simulink model "s_c_nbe_m32k"  (R2018a)
settings: Solver=VariableStepDiscrete  StartTime=0.0  StopTime=1000  RelTol=1e-3
undefined symbols (not defined in the file): fft_stages, n_taps, output_bits, pfb_coeff_gen_calc, xengbits
libraries: xbsIndex_r4 x23714, casper_library_misc x17, xps_library x4, casper_library_scopes x4, xbsReplacements_r4 x4
(part 4 of 171)

== system s_c_nbe_m32k/DDC ==
  note: DDS 18.17
  note: Mixer
  note: Filter
  sync : Inport
  dvalid : Inport  Port=2
  pol0_data : Inport  Port=3
  osc0 : Inport  Port=4
  pol1_data : Inport  Port=5
  osc1 : Inport  Port=6
  Assert : xbsIndex_r4/Assert  assert_type=on  type_source=Explicitly  gui_display_data_type=Boolean  arith_type=Boolean  n_bits=16  bin_pt=14  preci_type=Single  exp_width=8  frac_width=24  assert_rate=off  rate_source=Explicitly  period=1  output_port=on  block_type=assert
  Concat : xbsIndex_r4/Concat  num_inputs=2  dbl_ovrd=off  block_type=concat
  Concat1 : xbsIndex_r4/Concat  num_inputs=2  dbl_ovrd=off  block_type=concat
  Constant : xbsIndex_r4/Constant  const=0  gui_display_data_type=Fixed-point  arith_type=Unsigned  n_bits=1  bin_pt=0  preci_type=Single  exp_width=8  frac_width=24  explicit_period=on  period=1  equ=P=C  opselect=C  inp2=PCIN>>17  opr=+  inp1=P  carry=CIN  dbl_ovrd=off  block_type=constant
  Counter1 : xbsIndex_r4/Counter  cnt_type=Free Running  cnt_to=Inf  operation=Up  start_count=0  cnt_by_val=1  arith_type=Unsigned  n_bits=8  bin_pt=0  load_pin=off  rst=on  en=on  explicit_period=on  period=1  use_behavioral_HDL=off  implementation=DSP48  dbl_ovrd=off  block_type=counter
      settings: block_version=11.4
  Counter3 : xbsIndex_r4/Counter  cnt_type=Free Running  cnt_to=Inf  operation=Up  start_count=0  cnt_by_val=1  arith_type=Unsigned  n_bits=8  bin_pt=0  load_pin=off  rst=on  en=on  explicit_period=on  period=1  use_behavioral_HDL=off  implementation=DSP48  dbl_ovrd=off  block_type=counter
      settings: block_version=11.4
  Delay1 : xbsIndex_r4/Delay  rst=off  infoeditControl=Selection of Reset will increase slice count due to use of real FFs and instead of SRLs  en=off  latency=12  reg_retiming=off  dbl_ovrd=off  block_type=delay
  Delay2 : xbsIndex_r4/Delay  rst=off  infoeditControl=Selection of Reset will increase slice count due to use of real FFs and instead of SRLs  en=off  latency=12  reg_retiming=off  dbl_ovrd=off  block_type=delay
  Delay3 : xbsIndex_r4/Delay  rst=off  infoeditControl=Selection of Reset will increase slice count due to use of real FFs and instead of SRLs  en=off  latency=1  reg_retiming=off  dbl_ovrd=off  block_type=delay
      settings: infoedit=Hardware notes: A delay line is a chain, each link of which is an SRL16 or SRL32 followed by a flip-flop.
  Delay5 : xbsIndex_r4/Delay  rst=off  infoeditControl=Selection of Reset will increase slice count due to use of real FFs and instead of SRLs  en=off  latency=1  reg_retiming=off  dbl_ovrd=off  block_type=delay
      settings: infoedit=Hardware notes: A delay line is a chain, each link of which is an SRL16 or SRL32 followed by a flip-flop.
  Delay7 : xbsIndex_r4/Delay  rst=off  infoeditControl=Selection of Reset will increase slice count due to use of real FFs and instead of SRLs  en=off  latency=1  reg_retiming=off  dbl_ovrd=off  block_type=delay
      settings: infoedit=Hardware notes: A delay line is a chain, each link of which is an SRL16 or SRL32 followed by a flip-flop.
  Inverter : xbsIndex_r4/Inverter  en=off  latency=0  dbl_ovrd=off  block_type=inv
  Logical : xbsIndex_r4/Logical  Commented=on  logical_function=OR  inputs=2  en=off  latency=0  precision=Full  arith_type=Unsigned  n_bits=16  bin_pt=0  align_bp=on  dbl_ovrd=off  block_type=logical
  Register1 : xbsIndex_r4/Register  init=0  rst=on  en=on  dbl_ovrd=off  block_type=register
  bus_expand : Subsystem  mask(bus_expand){mode=divisions of equal size, outputNum=2, outputWidth=1, outputBinaryPt=0, outputArithmeticType=2, show_format=off, outputToWorkspace=off, variablePrefix=out, outputToModelAsWell=on}
      mask prompts: outputNum "Number of outputs:"; outputWidth "Output width:"; outputBinaryPt "Output binary point position:"; outputArithmeticType "Output arithmetic type (ufix=0, fix=1, bool=2):"; show_format "Print format string?"; outputToWorkspace "Output to workspace?"; variablePrefix "Variable name prefix:"; outputToModelAsWell "Output to model as well?"
      mask help:
      | Expands a 'bus' made using a bus_create or Xilinx
      | concat block.
      | The input will be divided into the specified number
      | of outputs with the specified arithmetic types.
      | Divisions are made from most significant bit.
      mask init: same as s_c_nbe_m32k/bus_expand1
      settings: AttributesFormatString=2 outputs
      mask TypeOptions mode: divisions of equal size | divisions of arbitrary size
      mask Callback mode: bus_expand_callback();
      mask Callback outputWidth: bus_expand_callback();
      mask Callback outputToWorkspace: bus_expand_callback();
  bus_expand10 : Subsystem  mask(bus_expand){mode=divisions of equal size, outputNum=16, outputWidth=18, outputBinaryPt=17, outputArithmeticType=1, show_format=off, outputToWorkspace=off, variablePrefix=Sin, outputToModelAsWell=off}
      mask prompts: outputNum "Number of outputs:"; outputWidth "Output width:"; outputBinaryPt "Output binary point position:"; outputArithmeticType "Output arithmetic type (ufix=0, fix=1, bool=2):"; show_format "Print format string?"; outputToWorkspace "Output to workspace?"; variablePrefix "Variable name prefix:"; outputToModelAsWell "Output to model as well?"
      mask help:
      | Expands a 'bus' made using a bus_create or Xilinx
      | concat block.
      | The input will be divided into the specified number
      | of outputs with the specified arithmetic types.
      | Divisions are made from most significant bit.
      mask init: same as s_c_nbe_m32k/bus_expand1
      settings: AttributesFormatString=16 outputs
      mask TypeOptions mode: divisions of equal size | divisions of arbitrary size
      mask Callback mode: bus_expand_callback();
      mask Callback outputWidth: bus_expand_callback();
      mask Callback outputToWorkspace: bus_expand_callback();
  bus_expand5 : Subsystem  mask(bus_expand){mode=divisions of equal size, outputNum=16, outputWidth=18, outputBinaryPt=17, outputArithmeticType=1, show_format=off, outputToWorkspace=off, variablePrefix=Sin, outputToModelAsWell=off}
      mask prompts: outputNum "Number of outputs:"; outputWidth "Output width:"; outputBinaryPt "Output binary point position:"; outputArithmeticType "Output arithmetic type (ufix=0, fix=1, bool=2):"; show_format "Print format string?"; outputToWorkspace "Output to workspace?"; variablePrefix "Variable name prefix:"; outputToModelAsWell "Output to model as well?"
      mask help:
      | Expands a 'bus' made using a bus_create or Xilinx
      | concat block.
      | The input will be divided into the specified number
      | of outputs with the specified arithmetic types.
      | Divisions are made from most significant bit.
      mask init: same as s_c_nbe_m32k/bus_expand1
      settings: AttributesFormatString=16 outputs
      mask TypeOptions mode: divisions of equal size | divisions of arbitrary size
      mask Callback mode: bus_expand_callback();
      mask Callback outputWidth: bus_expand_callback();
      mask Callback outputToWorkspace: bus_expand_callback();
  bus_expand6 : Subsystem  mask(bus_expand){mode=divisions of equal size, outputNum=16, outputWidth=18, outputBinaryPt=17, outputArithmeticType=1, show_format=off, outputToWorkspace=off, variablePrefix=Sin, outputToModelAsWell=off}
      mask prompts: outputNum "Number of outputs:"; outputWidth "Output width:"; outputBinaryPt "Output binary point position:"; outputArithmeticType "Output arithmetic type (ufix=0, fix=1, bool=2):"; show_format "Print format string?"; outputToWorkspace "Output to workspace?"; variablePrefix "Variable name prefix:"; outputToModelAsWell "Output to model as well?"
      mask help:
      | Expands a 'bus' made using a bus_create or Xilinx
      | concat block.
      | The input will be divided into the specified number
      | of outputs with the specified arithmetic types.
      | Divisions are made from most significant bit.
      mask init: same as s_c_nbe_m32k/bus_expand1
      settings: AttributesFormatString=16 outputs
      mask TypeOptions mode: divisions of equal size | divisions of arbitrary size
      mask Callback mode: bus_expand_callback();
      mask Callback outputWidth: bus_expand_callback();
      mask Callback outputToWorkspace: bus_expand_callback();
  bus_expand9 : Subsystem  mask(bus_expand){mode=divisions of equal size, outputNum=16, outputWidth=18, outputBinaryPt=17, outputArithmeticType=1, show_format=off, outputToWorkspace=off, variablePrefix=Sin, outputToModelAsWell=off}
      mask prompts: outputNum "Number of outputs:"; outputWidth "Output width:"; outputBinaryPt "Output binary point position:"; outputArithmeticType "Output arithmetic type (ufix=0, fix=1, bool=2):"; show_format "Print format string?"; outputToWorkspace "Output to workspace?"; variablePrefix "Variable name prefix:"; outputToModelAsWell "Output to model as well?"
      mask help:
      | Expands a 'bus' made using a bus_create or Xilinx
      | concat block.
      | The input will be divided into the specified number
      | of outputs with the specified arithmetic types.
      | Divisions are made from most significant bit.
      mask init: same as s_c_nbe_m32k/bus_expand1
      settings: AttributesFormatString=16 outputs
      mask TypeOptions mode: divisions of equal size | divisions of arbitrary size
      mask Callback mode: bus_expand_callback();
      mask Callback outputWidth: bus_expand_callback();
      mask Callback outputToWorkspace: bus_expand_callback();
  bus_mult : Subsystem  mask(bus_mult){n_bits_a=[10,10,10,10,10,10,10,10], bin_pt_a=9, type_a=1, cmplx_a=on, n_bits_b=[18,18,18,18,18,18,18,18], bin_pt_b=17, type_b=1, cmplx_b=on, misc=on, floating_point=off, float_type=single, input_vec_a=1, input_vec_b=1, frac_width=19, exp_width=6, n_bits_out=18, bin_pt_out=17, type_out=1, quantization=1, overflow=0, mult_latency=7, add_latency=7, conv_latency=7, max_fanout=1, fan_latency=3, multiplier_implementation=embedded multiplier core, pipeline_cmult_en=off, pipeline_latency=0}
      mask prompts: n_bits_a "a input bit widths"; bin_pt_a "a input binary points"; type_a "a input type (Unsigned=0, Signed=1)"; cmplx_a "a input complex"; n_bits_b "b input bit widths"; bin_pt_b "b input binary points"; type_b "b input type (Unsigned=0, Signed=1)"; cmplx_b "b input complex"; misc "misc support"; floating_point "floating point"; float_type "float type"; input_vec_a "a input vector in bus"; input_vec_b "b input vector in bus"; frac_width "fraction width"; exp_width "exponent width"; n_bits_out "output bit widths"; bin_pt_out "output binary points"; type_out "output type (Unsigned=0, Signed=1)"; quantization "quantization strategy (Truncate=0, Round  (unbiased: +/- Inf)=1)"; overflow "overflow strategy (Wrap=0, Saturate=1, Flag as error=2)"; mult_latency "multiplier latency"; add_latency "adder latency"; conv_latency "convert latency"; max_fanout "limit fanout to ?"; fan_latency "fanout register latency"; multiplier_implementation "multiplier implementation"; pipeline_cmult_en "pipeline complex mult"; pipeline_latency "pipeline latency"
      mask help: Multiply components of two busses
      mask init:
      | bus_mult_init(gcb, ...
      |     'n_bits_a', n_bits_a, ...
      |     'bin_pt_a', bin_pt_a, ...
      |     'type_a', type_a, ...
      |     'cmplx_a', cmplx_a, ...
      |     'n_bits_b', n_bits_b, ...
      |     'bin_pt_b', bin_pt_b, ...
      |     'type_b', type_b, ...
      |     'cmplx_b', cmplx_b, ...
      |     'n_bits_out', n_bits_out, ...
      |     'bin_pt_out', bin_pt_out, ...
      |     'type_out', type_out, ...
      |     'floating_point', floating_point, ...
      |     'float_type', float_type, ...
      |     'exp_width', exp_width, ...
      |     'input_vec_a', input_vec_a, ...
      |     'input_vec_b', input_vec_b, ...
      |     'frac_width', frac_width, ...         
      |     'quantization', quantization, ...
      |     'overflow', overflow, ...
      |     'mult_latency', mult_latency, ...
      |     'add_latency', add_latency, ...
      |     'conv_latency', conv_latency, ...
      |     'max_fanout', max_fanout, ...
      |     'pipeline_cmult_en', pipeline_cmult_en, ...
      |     'pipeline_latency', pipeline_latency, ...
      |     'fan_latency', fan_latency, ...
      |     'multiplier_implementation', multiplier_implementation, ...
      |     'misc', misc);
      mask Callback floating_point:
      | onoff = get_param(gcb, 'floating_point');
      | if strcmp(onoff,'on')
      |     enable_fixpt = 'off'
      |     set_param_state(gcb, 'float_type', 'on')
      | 
      |     set_param_state(gcb, 'input_vec_a', 'on')
      |     set_param_state(gcb, 'input_vec_b', 'on')
      | 
      |     f_type = get_param(gcb, 'float_type')
      |     if strcmp(f_type,'custom')
      |         set_param_state(gcb, 'exp_width', 'on')
      |         set_param_state(gcb, 'frac_width', 'on')
      |     else
      |         set_param_state(gcb, 'exp_width', 'off')
      |         set_param_state(gcb, 'frac_width', 'off')
      |     end
      | 
      | else
      |     enable_fixpt = 'on'
      |     set_param_state(gcb, 'float_type', 'off')
      |     set_param_state(gcb, 'exp_width', 'off')
      |     set_param_state(gcb, 'frac_width', 'off')
      |     set_param_state(gcb, 'input_vec_a', 'off')
      |     set_param_state(gcb, 'input_vec_b', 'off')
      | end
      | 
      | set_param_state(gcb, 'n_bits_a', enable_fixpt)
      | set_param_state(gcb, 'bin_pt_a', enable_fixpt)
      | set_param_state(gcb, 'type_a', enable_fixpt)
      | set_param_state(gcb, 'n_bits_b', enable_fixpt)
      | set_param_state(gcb, 'bin_pt_b', enable_fixpt)
      | set_param_state(gcb, 'type_b', enable_fixpt)
      | 
      | set_param_state(gcb, 'n_bits_out', enable_fixpt)
      | set_param_state(gcb, 'bin_pt_out', enable_fixpt)
      | set_param_state(gcb, 'type_out', enable_fixpt)
      | set_param_state(gcb, 'quantization', enable_fixpt)
      | set_param_state(gcb, 'overflow', enable_fixpt)
      mask TypeOptions float_type: single | custom
      mask Callback float_type:
      | f_type = get_param(gcb, 'float_type')
      | if strcmp(f_type,'custom')
      |     set_param_state(gcb, 'exp_width', 'on')
      |     set_param_state(gcb, 'frac_width', 'on')
      | else
      |     set_param_state(gcb, 'exp_width', 'off')
      |     set_param_state(gcb, 'frac_width', 'off')
      | end
      mask TypeOptions multiplier_implementation: behavioral HDL | standard core | embedded multiplier core
      mask Callback pipeline_cmult_en:
      | pipeline_en = get_param(gcb, 'pipeline_cmult_en');
      | if strcmp(pipeline_en,'on')
      | 
      |     set_param_state(gcb, 'pipeline_latency', 'on')
      | else
      |     set_param_state(gcb, 'pipeline_latency', 'off')
      | end
  bus_mult1 : Subsystem  mask(bus_mult){n_bits_a=[10,10,10,10,10,10,10,10], bin_pt_a=9, type_a=1, cmplx_a=on, n_bits_b=[18,18,18,18,18,18,18,18], bin_pt_b=17, type_b=1, cmplx_b=on, misc=off, floating_point=off, float_type=single, input_vec_a=1, input_vec_b=1, frac_width=19, exp_width=6, n_bits_out=18, bin_pt_out=17, type_out=1, quantization=1, overflow=0, mult_latency=7, add_latency=7, conv_latency=7, max_fanout=1, fan_latency=3, multiplier_implementation=embedded multiplier core, pipeline_cmult_en=off, pipeline_latency=0}
      mask prompts: n_bits_a "a input bit widths"; bin_pt_a "a input binary points"; type_a "a input type (Unsigned=0, Signed=1)"; cmplx_a "a input complex"; n_bits_b "b input bit widths"; bin_pt_b "b input binary points"; type_b "b input type (Unsigned=0, Signed=1)"; cmplx_b "b input complex"; misc "misc support"; floating_point "floating point"; float_type "float type"; input_vec_a "a input vector in bus"; input_vec_b "b input vector in bus"; frac_width "fraction width"; exp_width "exponent width"; n_bits_out "output bit widths"; bin_pt_out "output binary points"; type_out "output type (Unsigned=0, Signed=1)"; quantization "quantization strategy (Truncate=0, Round  (unbiased: +/- Inf)=1)"; overflow "overflow strategy (Wrap=0, Saturate=1, Flag as error=2)"; mult_latency "multiplier latency"; add_latency "adder latency"; conv_latency "convert latency"; max_fanout "limit fanout to ?"; fan_latency "fanout register latency"; multiplier_implementation "multiplier implementation"; pipeline_cmult_en "pipeline complex mult"; pipeline_latency "pipeline latency"
      mask help: Multiply components of two busses
      mask init: same as s_c_nbe_m32k/DDC/bus_mult
      mask Callback floating_point:
      | onoff = get_param(gcb, 'floating_point');
      | if strcmp(onoff,'on')
      |     enable_fixpt = 'off'
      |     set_param_state(gcb, 'float_type', 'on')
      | 
      |     set_param_state(gcb, 'input_vec_a', 'on')
      |     set_param_state(gcb, 'input_vec_b', 'on')
      | 
      |     f_type = get_param(gcb, 'float_type')
      |     if strcmp(f_type,'custom')
      |         set_param_state(gcb, 'exp_width', 'on')
      |         set_param_state(gcb, 'frac_width', 'on')
      |     else
      |         set_param_state(gcb, 'exp_width', 'off')
      |         set_param_state(gcb, 'frac_width', 'off')
      |     end
      | 
      | else
      |     enable_fixpt = 'on'
      |     set_param_state(gcb, 'float_type', 'off')
      |     set_param_state(gcb, 'exp_width', 'off')
      |     set_param_state(gcb, 'frac_width', 'off')
      |     set_param_state(gcb, 'input_vec_a', 'off')
      |     set_param_state(gcb, 'input_vec_b', 'off')
      | end
      | 
      | set_param_state(gcb, 'n_bits_a', enable_fixpt)
      | set_param_state(gcb, 'bin_pt_a', enable_fixpt)
      | set_param_state(gcb, 'type_a', enable_fixpt)
      | set_param_state(gcb, 'n_bits_b', enable_fixpt)
      | set_param_state(gcb, 'bin_pt_b', enable_fixpt)
      | set_param_state(gcb, 'type_b', enable_fixpt)
      | 
      | set_param_state(gcb, 'n_bits_out', enable_fixpt)
      | set_param_state(gcb, 'bin_pt_out', enable_fixpt)
      | set_param_state(gcb, 'type_out', enable_fixpt)
      | set_param_state(gcb, 'quantization', enable_fixpt)
      | set_param_state(gcb, 'overflow', enable_fixpt)
      mask TypeOptions float_type: single | custom
      mask Callback float_type:
      | f_type = get_param(gcb, 'float_type')
      | if strcmp(f_type,'custom')
      |     set_param_state(gcb, 'exp_width', 'on')
      |     set_param_state(gcb, 'frac_width', 'on')
      | else
      |     set_param_state(gcb, 'exp_width', 'off')
      |     set_param_state(gcb, 'frac_width', 'off')
      | end
      mask TypeOptions multiplier_implementation: behavioral HDL | standard core | embedded multiplier core
      mask Callback pipeline_cmult_en:
      | pipeline_en = get_param(gcb, 'pipeline_cmult_en');
      | if strcmp(pipeline_en,'on')
      | 
      |     set_param_state(gcb, 'pipeline_latency', 'on')
      | else
      |     set_param_state(gcb, 'pipeline_latency', 'off')
      | end
  convert_of : Subsystem  Commented=on  AncestorBlock=casper_library_misc/convert_of  mask(convert_of){bit_width_i=44, binary_point_i=34, bit_width_o=18, binary_point_o=17, latency=2, overflow=Saturate, quantization=Round  (unbiased: +/- Inf)}
      mask prompts: bit_width_i "Bit Width In"; binary_point_i "Binary Point In"; bit_width_o "Bit Width Out"; binary_point_o "Binary Point Out"; overflow "Overflow Behaviour"; quantization "Quantization Behaviour"
      mask help:
      | Converts from one 2's complement bit-width
      | and/or binary point position to another.
      | Includes underflow/overflow indicator.
      mask init:
      | convert_of_init(gcb, ...
      |     'bit_width_i', bit_width_i, ...
      |     'binary_point_i', binary_point_i, ...
      |     'bit_width_o', bit_width_o, ...
      |     'binary_point_o', binary_point_o, ...
      |     'latency', latency, ...
      |     'overflow', overflow, ...
      |     'quantization', quantization);
      settings: AttributesFormatString=[44,34]->[18,17]
      mask TypeOptions overflow: Wrap | Saturate | Error
      mask TypeOptions quantization: Truncate | Round  (unbiased: +/- Inf) | Round  (unbiased: even values)
  convert_of1 : Subsystem  Commented=on  AncestorBlock=casper_library_misc/convert_of  mask(convert_of){bit_width_i=44, binary_point_i=34, bit_width_o=18, binary_point_o=17, latency=2, overflow=Saturate, quantization=Round  (unbiased: +/- Inf)}
      mask prompts: bit_width_i "Bit Width In"; binary_point_i "Binary Point In"; bit_width_o "Bit Width Out"; binary_point_o "Binary Point Out"; overflow "Overflow Behaviour"; quantization "Quantization Behaviour"
      mask help:
      | Converts from one 2's complement bit-width
      | and/or binary point position to another.
      | Includes underflow/overflow indicator.
      mask init: same as s_c_nbe_m32k/DDC/convert_of
      settings: AttributesFormatString=[44,34]->[18,17]
      mask TypeOptions overflow: Wrap | Saturate | Error
      mask TypeOptions quantization: Truncate | Round  (unbiased: +/- Inf) | Round  (unbiased: even values)
  ddc_in_sync_cnt : Subsystem  Tag=xps:sw_reg  AncestorBlock=xps_library/Memory/software_register  mask(swreg){io_dir=To Processor, io_delay=0, init_val=0, sample_period=1, names=reg, bitwidths=8, bin_pts=0, arith_types=0, sim_port=off, show_format=on}
      mask prompts: io_dir "I/O direction"; io_delay "I/O delay"; init_val "Initial Value"; sample_period "Sample period"; names "Bitfield names [msb...lsb]"; bitwidths "Bitfield widths"; bin_pts "Bitfield binary pts"; arith_types "Bitfield types, ufix=0, fix=1, bool=2"; sim_port "Provide sim input/output?"; show_format "Print format string?"
      mask help: A 32-bit software-accessible register. Can be divided into bitfields of varying widths and types using the fields in the block mask.
      mask init:
      | swreg_init(gcb)
      settings: AttributesFormatString=1output:uf8.0 = 8 bits
      mask TypeOptions io_dir: To Processor | From Processor
      mask Callback io_dir:
      | mask_enables = get_param(gcb, 'MaskEnables');
      | mask_names = get_param(gcb, 'MaskNames');
      | if strcmp(get_param(gcb, 'io_dir'), 'To Processor'),
      |     mask_enables{ismember(mask_names, 'sample_period')} = 'off';
      | else
      |     mask_enables{ismember(mask_names, 'sample_period')} = 'on';
      | end
      | set_param(gcb, 'MaskEnables', mask_enables);
      mask DialogControl ParameterTabVar0 Prompt: Setup
  ddc_out_sync_cnt : Subsystem  Tag=xps:sw_reg  AncestorBlock=xps_library/Memory/software_register  mask(swreg){io_dir=To Processor, io_delay=0, init_val=0, sample_period=1, names=reg, bitwidths=8, bin_pts=0, arith_types=0, sim_port=off, show_format=on}
      mask prompts: io_dir "I/O direction"; io_delay "I/O delay"; init_val "Initial Value"; sample_period "Sample period"; names "Bitfield names [msb...lsb]"; bitwidths "Bitfield widths"; bin_pts "Bitfield binary pts"; arith_types "Bitfield types, ufix=0, fix=1, bool=2"; sim_port "Provide sim input/output?"; show_format "Print format string?"
      mask help: A 32-bit software-accessible register. Can be divided into bitfields of varying widths and types using the fields in the block mask.
      mask init:
      | swreg_init(gcb)
      settings: AttributesFormatString=1output:uf8.0 = 8 bits
      mask TypeOptions io_dir: To Processor | From Processor
      mask Callback io_dir:
      | mask_enables = get_param(gcb, 'MaskEnables');
      | mask_names = get_param(gcb, 'MaskNames');
      | if strcmp(get_param(gcb, 'io_dir'), 'To Processor'),
      |     mask_enables{ismember(mask_names, 'sample_period')} = 'off';
      | else
      |     mask_enables{ismember(mask_names, 'sample_period')} = 'on';
      | end
      | set_param(gcb, 'MaskEnables', mask_enables);
      mask DialogControl ParameterTabVar0 Prompt: Setup
  dec_fir_async1 : Subsystem  Tag=casper:dec_fir_async  AncestorBlock=casper_library_downconverter/dec_fir_async  mask(dec_fir_async){n_inputs=16, coeff=[-0.000309,-0.000234,-0.000315,-0.000409,-0.000513,-0.000626,-0.000747,-0.000870,-0.000994,-0.001113,-0.001222,-0.001316,-0.001388,-0.001433,-0.001444,-0.001415,-0.001343,-0.001221,-0.001046,-0.000817,-0.000533,-0.000195,0.000193,0.000628,0.001100,0.001602,0.002121,0.002645,0.003159,0.003646,0.004091,0.004475,0.004781,0.004993,0.005095,0.005074,0.004920,0.004623,0.004179,0.003589,0.002855,0.001988,0.001000,-0.000089,-0.001258,-0.002478,-0.003716,-0.004939,-0.006108,-0.007182,-0.008120,-0.008882,-0.009426,-0.009715,-0.009715,-0.009394,-0.008727,-0.007696,-0.006289,-0.004503,-0.002341,0.000182,0.003046,0.006221,0.009667,0.013340,0.017186,0.021147,0.025161,0.029161,0.033078,0.036845,0.040394,0.043661,0.046586,0.049113,0.051195,0.052792,0.053875,0.054421,0.054421,0.053875,0.052792,0.051195,0.049113,0.046586,0.043661,0.040394,0.036845,0.033078,0.029161,0.025161,0.021147,0.017186,0.013340,0.009667,0.006221,0.003046,0.000182,-0.002341,-0.004503,-0.006289,-0.007696,-0.008727,-0.009394,-0.009715,-0.009715,-0.009426,-0.008882,-0.008120,-0.007182,-0.006108,-0.004939,-0.003716,-0.002478,-0.001258,-0.000089,0.001000,0.001988,0.002855,0.003589,0.004179,0.004623,0.004920,0.005074,0.005095,0.004993,0.004781,0.004475,0.004091,0.003646,0.003159,0.002645,0.002121,0.001602,0.001100,0.000628,0.000193,-0.000195,-0.000533,-0.000817,-0.001046,-0.001221,-0.001343,-0.001415,-0.001444,-0.001433,-0.001388,-0.001316,-0.001222,-0.001113,-0.000994,-0.000870,-0.000747,-0.000626,-0.000513,-0.000409,-0.000315,-0.000234,-0.000309], output_width=18, output_bp=17, quantization=Round  (unbiased: +/- Inf), add_latency=7, mult_latency=7, conv_latency=7, coeff_bit_width=18, coeff_bin_pt=17, lshift=1, absorb_adders=on, adder_imp=DSP48, async=on, bus_input=off, input_width=0, input_bp=0, input_type=Signed}
      mask prompts: n_inputs "Number of Parallel Streams"; coeff "Coefficients"; output_width "Output bitwidth"; output_bp "Output binary point"; quantization "Quantization Behavior"; add_latency "Add Latency"; mult_latency "Mult Latency"; conv_latency "Convert latency"; coeff_bit_width "Coefficient bitwidth"; coeff_bin_pt "Coefficient binary point"; lshift "Post adder-tree shift"; absorb_adders "Absorb adders into DSP slices"; adder_imp "Adder implementation"; async "Asynchronous ops"; bus_input "Bus input"; input_width "Input bitwidth"; input_bp "Input binary point"; input_type "Input datatype"
      mask help: FIR filter which can handle multiple time samples in parallel and decimates down to 1 time sample. If coefficients are symmetric, will automatically fold before multiplying.
      mask init:
      | dec_fir_async_init(gcb);
      settings: AttributesFormatString=|
      | 160 taps
      | 18_17 r/i
      mask TypeOptions quantization: Truncate | Round  (unbiased: +/- Inf) | Round  (unbiased: Even Values)
      mask TypeOptions adder_imp: Behavioral | Fabric | DSP48
      mask Callback bus_input:
      | onoff = get_param(gcb, 'bus_input');
      | set_param_state(gcb, 'input_width', onoff)
      | set_param_state(gcb, 'input_bp', onoff)
      | set_param_state(gcb, 'input_type', onoff)
      mask TypeOptions input_type: Signed | Unsigned
  dec_fir_async3 : Subsystem  Tag=casper:dec_fir_async  AncestorBlock=casper_library_downconverter/dec_fir_async  mask(dec_fir_async){n_inputs=16, coeff=[-0.000309,-0.000234,-0.000315,-0.000409,-0.000513,-0.000626,-0.000747,-0.000870,-0.000994,-0.001113,-0.001222,-0.001316,-0.001388,-0.001433,-0.001444,-0.001415,-0.001343,-0.001221,-0.001046,-0.000817,-0.000533,-0.000195,0.000193,0.000628,0.001100,0.001602,0.002121,0.002645,0.003159,0.003646,0.004091,0.004475,0.004781,0.004993,0.005095,0.005074,0.004920,0.004623,0.004179,0.003589,0.002855,0.001988,0.001000,-0.000089,-0.001258,-0.002478,-0.003716,-0.004939,-0.006108,-0.007182,-0.008120,-0.008882,-0.009426,-0.009715,-0.009715,-0.009394,-0.008727,-0.007696,-0.006289,-0.004503,-0.002341,0.000182,0.003046,0.006221,0.009667,0.013340,0.017186,0.021147,0.025161,0.029161,0.033078,0.036845,0.040394,0.043661,0.046586,0.049113,0.051195,0.052792,0.053875,0.054421,0.054421,0.053875,0.052792,0.051195,0.049113,0.046586,0.043661,0.040394,0.036845,0.033078,0.029161,0.025161,0.021147,0.017186,0.013340,0.009667,0.006221,0.003046,0.000182,-0.002341,-0.004503,-0.006289,-0.007696,-0.008727,-0.009394,-0.009715,-0.009715,-0.009426,-0.008882,-0.008120,-0.007182,-0.006108,-0.004939,-0.003716,-0.002478,-0.001258,-0.000089,0.001000,0.001988,0.002855,0.003589,0.004179,0.004623,0.004920,0.005074,0.005095,0.004993,0.004781,0.004475,0.004091,0.003646,0.003159,0.002645,0.002121,0.001602,0.001100,0.000628,0.000193,-0.000195,-0.000533,-0.000817,-0.001046,-0.001221,-0.001343,-0.001415,-0.001444,-0.001433,-0.001388,-0.001316,-0.001222,-0.001113,-0.000994,-0.000870,-0.000747,-0.000626,-0.000513,-0.000409,-0.000315,-0.000234,-0.000309], output_width=18, output_bp=17, quantization=Round  (unbiased: +/- Inf), add_latency=7, mult_latency=7, conv_latency=7, coeff_bit_width=18, coeff_bin_pt=17, lshift=1, absorb_adders=on, adder_imp=DSP48, async=on, bus_input=off, input_width=0, input_bp=0, input_type=Signed}
      mask prompts: n_inputs "Number of Parallel Streams"; coeff "Coefficients"; output_width "Output bitwidth"; output_bp "Output binary point"; quantization "Quantization Behavior"; add_latency "Add Latency"; mult_latency "Mult Latency"; conv_latency "Convert latency"; coeff_bit_width "Coefficient bitwidth"; coeff_bin_pt "Coefficient binary point"; lshift "Post adder-tree shift"; absorb_adders "Absorb adders into DSP slices"; adder_imp "Adder implementation"; async "Asynchronous ops"; bus_input "Bus input"; input_width "Input bitwidth"; input_bp "Input binary point"; input_type "Input datatype"
      mask help: FIR filter which can handle multiple time samples in parallel and decimates down to 1 time sample. If coefficients are symmetric, will automatically fold before multiplying.
      mask init:
      | dec_fir_async_init(gcb);
      settings: AttributesFormatString=|
      | 160 taps
      | 18_17 r/i
      mask TypeOptions quantization: Truncate | Round  (unbiased: +/- Inf) | Round  (unbiased: Even Values)
      mask TypeOptions adder_imp: Behavioral | Fabric | DSP48
      mask Callback bus_input:
      | onoff = get_param(gcb, 'bus_input');
      | set_param_state(gcb, 'input_width', onoff)
      | set_param_state(gcb, 'input_bp', onoff)
      | set_param_state(gcb, 'input_type', onoff)
      mask TypeOptions input_type: Signed | Unsigned
  edge_detect2 : Subsystem  mask(edge_detect){edge=Rising, polarity=Active High, x_in=[0 0.08 0.08 0.16 0.16 0.24 0.24 0.32 0.32 0.4], y_in=[-1 -1  1  1  1  1  1  1  1  1], x_out=[0.6 0.68 0.68 0.76 0.76 0.84 0.84 0.92 0.92 1], y_out=[-1 -1  1  1 -1 -1 -1 -1 -1 -1]}
      mask prompts: edge "Edge Type"; polarity "Output Polarity"; x_in "Input X Positions"; y_in "Input Y Positions"; x_out "Output X Positions"; y_out "Output Y Positions"
      mask help: Output is active for one-cycle after each edge of the specified type (i.e. rising, falling or both).
      mask init: same as s_c_nbe_m32k/edge_detect1
      settings: AttributesFormatString=|
      | rising edges
      | active high
      mask Help: Output is active for one-cycle after each edge of the specified type (i.e. rising, falling, or both).  Latency is zero.
      mask TypeOptions edge: Rising | Falling | Both
      mask TypeOptions polarity: Active High | Active Low
      mask Display:
      | plot(x_in_num,0.5+y_in_num*0.2);
      | plot(x_out_num,0.5+y_out_num*0.2);
  edge_detect3 : Subsystem  mask(edge_detect){edge=Rising, polarity=Active High, x_in=[0 0.08 0.08 0.16 0.16 0.24 0.24 0.32 0.32 0.4], y_in=[-1 -1  1  1  1  1  1  1  1  1], x_out=[0.6 0.68 0.68 0.76 0.76 0.84 0.84 0.92 0.92 1], y_out=[-1 -1  1  1 -1 -1 -1 -1 -1 -1]}
      mask prompts: edge "Edge Type"; polarity "Output Polarity"; x_in "Input X Positions"; y_in "Input Y Positions"; x_out "Output X Positions"; y_out "Output Y Positions"
      mask help: Output is active for one-cycle after each edge of the specified type (i.e. rising, falling or both).
      mask init: same as s_c_nbe_m32k/edge_detect1
      settings: AttributesFormatString=|
      | rising edges
      | active high
      mask Help: Output is active for one-cycle after each edge of the specified type (i.e. rising, falling, or both).  Latency is zero.
      mask TypeOptions edge: Rising | Falling | Both
      mask TypeOptions polarity: Active High | Active Low
      mask Display:
      | plot(x_in_num,0.5+y_in_num*0.2);
      | plot(x_out_num,0.5+y_out_num*0.2);
  pipeline21 : Subsystem  Tag=cmac_delinked  mask(pipeline){csp_latency=2}
      mask prompts: csp_latency "Latency"
      mask help:
      | An explicitly laid-out delay line to avoid mapping to SRL16s
      | for use in pipelining to help achieve timing closure.
      mask init:
      | pipeline_init(gcb,'latency',csp_latency);
      settings: AttributesFormatString=Latency = %<latency>
      mask Display:
      | port_label('input', 1, 'd');
      | port_label('output', 1, 'q');
      | disp(['Z^-', num2str(csp_latency)]);
  pipeline22 : Subsystem  Tag=cmac_delinked  mask(pipeline){csp_latency=2}
      mask prompts: csp_latency "Latency"
      mask help:
      | An explicitly laid-out delay line to avoid mapping to SRL16s
      | for use in pipelining to help achieve timing closure.
      mask init:
      | pipeline_init(gcb,'latency',csp_latency);
      settings: AttributesFormatString=Latency = %<latency>
      mask Display:
      | port_label('input', 1, 'd');
      | port_label('output', 1, 'q');
      | disp(['Z^-', num2str(csp_latency)]);
  pipeline39 : Subsystem  Tag=cmac_delinked  mask(pipeline){csp_latency=2}
      mask prompts: csp_latency "Latency"
      mask help:
      | An explicitly laid-out delay line to avoid mapping to SRL16s
      | for use in pipelining to help achieve timing closure.
      mask init:
      | pipeline_init(gcb,'latency',csp_latency);
      settings: AttributesFormatString=Latency = %<latency>
      mask Display:
      | port_label('input', 1, 'd');
      | port_label('output', 1, 'q');
      | disp(['Z^-', num2str(csp_latency)]);
  pipeline40 : Subsystem  Tag=cmac_delinked  mask(pipeline){csp_latency=2}
      mask prompts: csp_latency "Latency"
      mask help:
      | An explicitly laid-out delay line to avoid mapping to SRL16s
      | for use in pipelining to help achieve timing closure.
      mask init:
      | pipeline_init(gcb,'latency',csp_latency);
      settings: AttributesFormatString=Latency = %<latency>
      mask Display:
      | port_label('input', 1, 'd');
      | port_label('output', 1, 'q');
      | disp(['Z^-', num2str(csp_latency)]);
  ri_to_c1 : casper_library_misc/ri_to_c  Commented=on
      settings: SourceProductName=CASPER DSP Blockset
  ddc_sync : Outport
  ddc_pol0 : Outport  Port=2
  ddc_pol1 : Outport  Port=3
  ddc_dv : Outport  Port=4
  ddc_of : Outport  Port=5
  tag scope: dec_dv=global, dec_sync=global, mix_80_0=global, mix_dvalid=global, mix_sync=global
  wires:
  bus_expand/1(msb_out2) -> [mix_sync]
  bus_expand/2(lsb_out1) -> [mix_dvalid]
  Concat/1 -> bus_mult/3(misci)
  bus_mult/2(misco) -> bus_expand/1(bus_in)
  [ddc_sync] -> ddc_sync/1
  [ddc_pol0] -> ddc_pol0/1
  [ddc_pol1] -> ddc_pol1/1
  pol0_data/1 -> bus_mult/1(a)
  osc0/1 -> bus_mult/2(b)
  pol1_data/1 -> bus_mult1/1(a)
  osc1/1 -> bus_mult1/2(b)
  bus_mult/1(a*b) -> [mix_80_0]
  bus_mult1/1(a*b) -> [mix_80_1]
  dvalid/1 -> Concat/2
  sync/1 -> Concat/1
  [cnt_rst] -> pipeline22/1(d)
  Counter1/1 -> ddc_out_sync_cnt/1(out_reg)
  pipeline21/1(q) -> Counter1/2
  pipeline22/1(q) -> Counter1/1
  [ddc_sync] -> pipeline21/1(d)
  [ddc_dvalid] -> ddc_dv/1
  Delay3/1 -> bus_expand5/1(bus_in)
  Delay5/1 -> bus_expand9/1(bus_in)
  bus_expand9/1(msb_out16) -> dec_fir_async1/3(real1)
  bus_expand9/2(out15) -> dec_fir_async1/4(imag1)
  bus_expand9/3(out14) -> dec_fir_async1/5(real2)
  bus_expand9/4(out13) -> dec_fir_async1/6(imag2)
  bus_expand9/5(out12) -> dec_fir_async1/7(real3)
  bus_expand9/6(out11) -> dec_fir_async1/8(imag3)
  bus_expand9/7(out10) -> dec_fir_async1/9(real4)
  bus_expand9/8(out9) -> dec_fir_async1/10(imag4)
  bus_expand9/9(out8) -> dec_fir_async1/11(real5)
  bus_expand9/10(out7) -> dec_fir_async1/12(imag5)
  bus_expand9/11(out6) -> dec_fir_async1/13(real6)
  bus_expand9/12(out5) -> dec_fir_async1/14(imag6)
  bus_expand9/13(out4) -> dec_fir_async1/15(real7)
  bus_expand9/14(out3) -> dec_fir_async1/16(imag7)
  bus_expand9/15(out2) -> dec_fir_async1/17(real8)
  bus_expand9/16(lsb_out1) -> dec_fir_async1/18(imag8)
  bus_expand10/1(msb_out16) -> dec_fir_async1/19(real9)
  bus_expand10/3(out14) -> dec_fir_async1/21(real10)
  bus_expand10/2(out15) -> dec_fir_async1/20(imag9)
  bus_expand10/4(out13) -> dec_fir_async1/22(imag10)
  bus_expand10/5(out12) -> dec_fir_async1/23(real11)
  bus_expand10/7(out10) -> dec_fir_async1/25(real12)
  bus_expand10/6(out11) -> dec_fir_async1/24(imag11)
  bus_expand10/8(out9) -> dec_fir_async1/26(imag12)
  bus_expand10/9(out8) -> dec_fir_async1/27(real13)
  bus_expand10/10(out7) -> dec_fir_async1/28(imag13)
  bus_expand10/11(out6) -> dec_fir_async1/29(real14)
  bus_expand10/12(out5) -> dec_fir_async1/30(imag14)
  bus_expand10/14(out3) -> dec_fir_async1/32(imag15)
  bus_expand10/13(out4) -> dec_fir_async1/31(real15)
  bus_expand10/15(out2) -> dec_fir_async1/33(real16)
  bus_expand10/16(lsb_out1) -> dec_fir_async1/34(imag16)
  dec_fir_async1/2(dout) -> Delay2/1
  [cnt_rst] -> pipeline40/1(d)
  Counter3/1 -> ddc_in_sync_cnt/1(out_reg)
  pipeline39/1(q) -> Counter3/2
  pipeline40/1(q) -> Counter3/1
  [dec_sync] -> pipeline39/1(d)
  [mix_dvalid] -> Register1/3
  Register1/1 -> edge_detect3/1(in), Inverter/1
  edge_detect3/1(out) -> [dec_dv]
  [dec_sync] -> dec_fir_async3/1(sync_in)
  [dec_dv] -> dec_fir_async1/2(dv_in)
  [dec_sync] -> dec_fir_async1/1(sync_in)
  [mix_80_1] -> Delay5/1, bus_expand10/1(bus_in)
  [mix_80_0] -> bus_expand6/1(bus_in), Delay3/1
  edge_detect2/1(out) -> [dec_sync]
  Inverter/1 -> Assert/1
  Assert/1 -> Register1/1
  [mix_sync] -> Delay7/1, Register1/2
  Delay7/1 -> edge_detect2/1(in)
  [ddc_of_pol0] -> Concat1/1
  [ddc_of_pol1] -> Concat1/2
  Concat1/1 -> ddc_of/1
  dec_fir_async3/2(dout) -> Delay1/1
  dec_fir_async3/1(sync_out) -> [ddc_sync]
  dec_fir_async3/3(dv_out) -> [ddc_dvalid]
  Constant/1 -> [ddc_of_pol1], [ddc_of_pol0]
  bus_expand6/16(lsb_out1) -> dec_fir_async3/34(imag16)
  bus_expand6/15(out2) -> dec_fir_async3/33(real16)
  bus_expand6/14(out3) -> dec_fir_async3/32(imag15)
  bus_expand6/13(out4) -> dec_fir_async3/31(real15)
  bus_expand6/12(out5) -> dec_fir_async3/30(imag14)
  bus_expand6/11(out6) -> dec_fir_async3/29(real14)
  bus_expand6/10(out7) -> dec_fir_async3/28(imag13)
  bus_expand6/9(out8) -> dec_fir_async3/27(real13)
  bus_expand6/8(out9) -> dec_fir_async3/26(imag12)
  bus_expand6/7(out10) -> dec_fir_async3/25(real12)
  bus_expand6/6(out11) -> dec_fir_async3/24(imag11)
  bus_expand6/5(out12) -> dec_fir_async3/23(real11)
  bus_expand6/4(out13) -> dec_fir_async3/22(imag10)
  bus_expand6/3(out14) -> dec_fir_async3/21(real10)
  bus_expand6/2(out15) -> dec_fir_async3/20(imag9)
  bus_expand6/1(msb_out16) -> dec_fir_async3/19(real9)
  bus_expand5/16(lsb_out1) -> dec_fir_async3/18(imag8)
  bus_expand5/15(out2) -> dec_fir_async3/17(real8)
  bus_expand5/14(out3) -> dec_fir_async3/16(imag7)
  bus_expand5/13(out4) -> dec_fir_async3/15(real7)
  bus_expand5/12(out5) -> dec_fir_async3/14(imag6)
  bus_expand5/11(out6) -> dec_fir_async3/13(real6)
  bus_expand5/10(out7) -> dec_fir_async3/12(imag5)
  bus_expand5/9(out8) -> dec_fir_async3/11(real5)
  bus_expand5/8(out9) -> dec_fir_async3/10(imag4)
  bus_expand5/7(out10) -> dec_fir_async3/9(real4)
  bus_expand5/6(out11) -> dec_fir_async3/8(imag3)
  bus_expand5/5(out12) -> dec_fir_async3/7(real3)
  bus_expand5/4(out13) -> dec_fir_async3/6(imag2)
  bus_expand5/3(out14) -> dec_fir_async3/5(real2)
  bus_expand5/2(out15) -> dec_fir_async3/4(imag1)
  bus_expand5/1(msb_out16) -> dec_fir_async3/3(real1)
  [dec_dv] -> dec_fir_async3/2(dv_in)
  convert_of1/1(dout) -> ri_to_c1/2
  convert_of/1(dout) -> ri_to_c1/1
  convert_of/2(of) -> Logical/1
  convert_of1/2(of) -> Logical/2
  Delay1/1 -> [ddc_pol0]
  Delay2/1 -> [ddc_pol1]

== system s_c_nbe_m32k/Subsystem ==
  time : Inport
  sync : Inport  Port=2
  dv : Inport  Port=3
  Delay15 : xbsIndex_r4/Delay  rst=off  infoeditControl=Selection of Reset will increase slice count due to use of real FFs and instead of SRLs  en=off  latency=1  reg_retiming=off  dbl_ovrd=off  block_type=delay
      settings: infoedit=Hardware notes: A delay line is a chain, each link of which is an SRL16 or SRL32 followed by a flip-flop.
  Delay16 : xbsIndex_r4/Delay  rst=off  infoeditControl=Selection of Reset will increase slice count due to use of real FFs and instead of SRLs  en=off  latency=1  reg_retiming=off  dbl_ovrd=off  block_type=delay
      settings: infoedit=Hardware notes: A delay line is a chain, each link of which is an SRL16 or SRL32 followed by a flip-flop.
  Register3 : xbsIndex_r4/Register  init=0  rst=on  en=on  dbl_ovrd=off  block_type=register
  Register7 : xbsIndex_r4/Register  init=0  rst=off  en=on  dbl_ovrd=off  block_type=register
  Register8 : xbsIndex_r4/Register  init=0  rst=off  en=on  dbl_ovrd=off  block_type=register
  Register9 : xbsIndex_r4/Register  init=0  rst=off  en=on  dbl_ovrd=off  block_type=register
  Slice35 : xbsIndex_r4/Slice  nbits=32  boolean_output=off  mode=Two Bit Locations  bit1=0  base1=MSB of Input  bit0=32  base0=LSB of Input  dbl_ovrd=off  block_type=slice
  Slice40 : xbsIndex_r4/Slice  nbits=32  boolean_output=off  mode=Lower Bit Location + Width  bit1=0  base1=MSB of Input  bit0=0  base0=LSB of Input  dbl_ovrd=off  block_type=slice
  edge_detect7 : Subsystem  mask(edge_detect){edge=Rising, polarity=Active High, x_in=[0 0.08 0.08 0.16 0.16 0.24 0.24 0.32 0.32 0.4], y_in=[-1 -1  1  1  1  1  1  1  1  1], x_out=[0.6 0.68 0.68 0.76 0.76 0.84 0.84 0.92 0.92 1], y_out=[-1 -1  1  1 -1 -1 -1 -1 -1 -1]}
      mask prompts: edge "Edge Type"; polarity "Output Polarity"; x_in "Input X Positions"; y_in "Input Y Positions"; x_out "Output X Positions"; y_out "Output Y Positions"
      mask help: Output is active for one-cycle after each edge of the specified type (i.e. rising, falling or both).
      mask init: same as s_c_nbe_m32k/edge_detect1
      settings: AttributesFormatString=|
      | rising edges
      | active high
      mask Help: Output is active for one-cycle after each edge of the specified type (i.e. rising, falling, or both).  Latency is zero.
      mask TypeOptions edge: Rising | Falling | Both
      mask TypeOptions polarity: Active High | Active Low
      mask Display:
      | plot(x_in_num,0.5+y_in_num*0.2);
      | plot(x_out_num,0.5+y_out_num*0.2);
  msw : Outport
  ls32 : Outport  Port=2
  wires:
  dv/1 -> Register7/2
  Register7/1 -> edge_detect7/1(in)
  Slice35/1 -> Delay15/1
  Delay15/1 -> Register8/1
  Register3/1 -> Register7/1
  Slice40/1 -> Delay16/1
  Register9/1 -> ls32/1
  edge_detect7/1(out) -> Register3/2, Register9/2, Register8/2
  Register8/1 -> msw/1
  Delay16/1 -> Register9/1
  sync/1 -> Register3/3, Register3/1
  time/1 -> Slice40/1, Slice35/1
